simulink model "Protection"  (R2023b)
settings: Solver=FixedStepDiscrete  StartTime=0.0  StopTime=10.0  FixedStep=1e-4  RelTol=1e-3
undefined symbols (not defined in the file): PROTECTION_STATUS
libraries: simulink x5
settings Model: DataDictionary=Protection.sldd  Creator=84339  LastModifiedBy=84339
settings OptimizationCC: DefaultParameterBehavior=Inlined  EnhancedBackFolding=on  PassReuseOutputArgsAs=Individual arguments  ZeroExternalMemoryAtStartup=off  ZeroInternalMemoryAtStartup=off  OptimizeBlockOrder=speed  DifferentSizesBufferReuse=on  OptimizationCustomize=off  EfficientTunableParamExpr=on
settings DebuggingCC: ParameterTunabilityLossMsg=error
settings SFSimCC: MATLABDynamicMemAlloc=off
settings RTWCC: Description=Embedded Coder  SystemTargetFile=ert.tlc  EmbeddedCoderDictionary=Arch.sldd  GenCodeOnly=on  TemplateMakefile=ert_default_tmf
settings CodeAppCC: ForceParamTrailComments=on  IgnoreCustomStorageClasses=off  OperatorAnnotations=on  SimulinkDataObjDesc=on  SFDataObjDesc=on  InsertBlockDesc=on
settings ERTTargetCC: TargetLangStandard=C99 (ISO)  GenerateSampleERTMain=on  InlinedParameterPlacement=NonHierarchical  ERTCustomFileTemplate=example_file_process.tlc

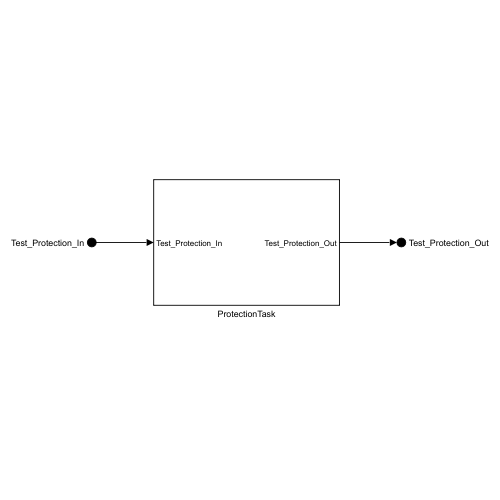
[thumbnail: Simulink's stored preview of the top-level diagram]
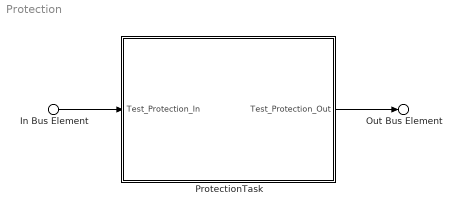
== system Protection ==
  In Bus Element : Inport  PortName=Test_Protection_In
  ProtectionTask : Subsystem
  Out Bus Element : Outport  PortName=Test_Protection_Out
  wires:
  In Bus Element/1 -> ProtectionTask/1(Test_Protection_In)
  ProtectionTask/1(Test_Protection_Out) -> Out Bus Element/1

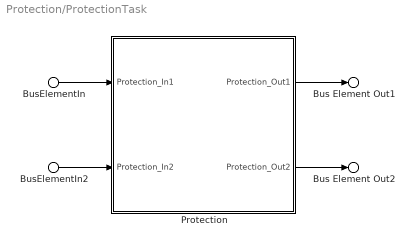
== system Protection/ProtectionTask ==
  BusElementIn : Inport  PortName=Test_Protection_In  Element=Protection_In1
  BusElementIn2 : Inport  PortName=Test_Protection_In  Element=Protection_In2
  Protection : Subsystem
  Bus Element Out1 : Outport  PortName=Test_Protection_Out  Element=Protection_Out1
  Bus Element Out2 : Outport  PortName=Test_Protection_Out  Element=Protection_Out2
  wires:
  BusElementIn/1 -> Protection/1(Protection_In1)
  Protection/1(Protection_Out1) -> Bus Element Out1/1
  BusElementIn2/1 -> Protection/2(Protection_In2)
  Protection/2(Protection_Out2) -> Bus Element Out2/1

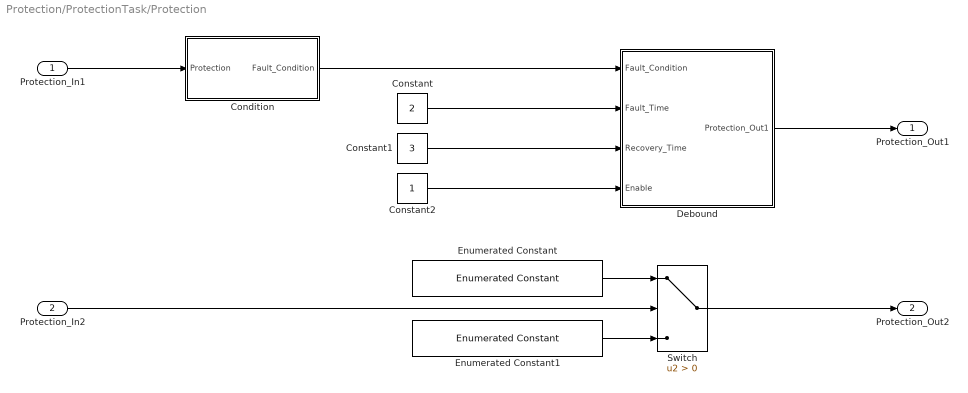
== system Protection/ProtectionTask/Protection ==
  Protection_In1 : Inport
  Protection_In2 : Inport  Port=2
  Condition : Subsystem
  Constant : Constant  Value=2  OutDataTypeStr=single
  Constant1 : Constant  Value=3  OutDataTypeStr=single
  Constant2 : Constant  OutDataTypeStr=boolean
  Debound : Subsystem
  Enumerated Constant : simulink/Sources/Enumerated Constant  OutDataTypeStr=Enum: PROTECTION_STATUS  Value=PROTECTION_STATUS.NORMAL  SampleTime=-1
  Enumerated Constant1 : simulink/Sources/Enumerated Constant  OutDataTypeStr=Enum: PROTECTION_STATUS  Value=PROTECTION_STATUS.ERROR  SampleTime=-1
  Switch : Switch  Criteria=u2 > Threshold  SaturateOnIntegerOverflow=off  InputSameDT=off
  Protection_Out1 : Outport
  Protection_Out2 : Outport  Port=2
  wires:
  Constant/1 -> Debound/2(Fault_Time)
  Constant1/1 -> Debound/3(Recovery_Time)
  Constant2/1 -> Debound/4(Enable)
  Debound/1(Protection_Out1) -> Protection_Out1/1
  Protection_In1/1 -> Condition/1(Protection)
  Condition/1(Fault_Condition) -> Debound/1(Fault_Condition)
  Protection_In2/1 -> Switch/2
  Enumerated Constant/1 -> Switch/1
  Enumerated Constant1/1 -> Switch/3
  Switch/1 -> Protection_Out2/1

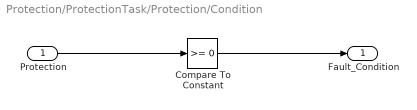
== system Protection/ProtectionTask/Protection/Condition ==
  Protection : Inport
  Compare To Constant : simulink/Logic and Bit Operations/Compare To Constant  relop=>=  const=0  OutDataTypeStr=boolean
  Fault_Condition : Outport
  wires:
  Compare To Constant/1 -> Fault_Condition/1
  Protection/1 -> Compare To Constant/1

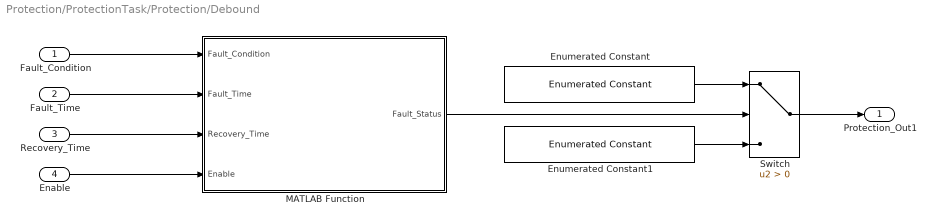
== system Protection/ProtectionTask/Protection/Debound ==
  Fault_Condition : Inport
  Fault_Time : Inport  Port=2
  Recovery_Time : Inport  Port=3
  Enable : Inport  Port=4
  Enumerated Constant : simulink/Sources/Enumerated Constant  OutDataTypeStr=Enum: PROTECTION_STATUS  Value=PROTECTION_STATUS.NORMAL  SampleTime=-1
  Enumerated Constant1 : simulink/Sources/Enumerated Constant  OutDataTypeStr=Enum: PROTECTION_STATUS  Value=PROTECTION_STATUS.ERROR  SampleTime=-1
  MATLAB Function : MATLAB Function  TreatAsAtomicUnit=on
  Switch : Switch  Criteria=u2 > Threshold  SaturateOnIntegerOverflow=off  InputSameDT=off
  Protection_Out1 : Outport
  wires:
  Enumerated Constant1/1 -> Switch/3
  MATLAB Function/1(Fault_Status) -> Switch/2
  Switch/1 -> Protection_Out1/1
  Enumerated Constant/1 -> Switch/1
  Fault_Condition/1 -> MATLAB Function/1(Fault_Condition)
  Fault_Time/1 -> MATLAB Function/2(Fault_Time)
  Recovery_Time/1 -> MATLAB Function/3(Recovery_Time)
  Enable/1 -> MATLAB Function/4(Enable)

== matlab function Protection/ProtectionTask/Protection/Debound/MATLAB Function ==
  data: Fault_Condition input; Fault_Status output; Fault_Time input; Recovery_Time input; Enable input
function Fault_Status = Debounce_Function(Fault_Condition, Fault_Time, Recovery_Time, Enable)
%#codegen

persistent Fault_Timer;
persistent Recovery_Timer;
persistent Fault_Active;

if isempty(Fault_Timer)
    Fault_Timer = single(0.0);
    Recovery_Timer = single(0.0);
    Fault_Active = false;
end

Ts = single(0.01);  % 10ms

if ~Enable
    Fault_Timer = single(0.0);
    Recovery_Timer = single(0.0);
    Fault_Active = false;

else
    if ~Fault_Active

        % Fault detection
        if Fault_Condition
            Fault_Timer = Fault_Timer + Ts;
        else
            Fault_Timer = single(0.0);
        end

        if Fault_Timer >= single(Fault_Time)
            Fault_Active = true;
            Recovery_Timer = single(0.0);
        end

    else

        % Fault recovery
        if ~Fault_Condition
            Recovery_Timer = Recovery_Timer + Ts;
        else
            Recovery_Timer = single(0.0);
        end

        if Recovery_Timer >= single(Recovery_Time)
            Fault_Active = false;
            Fault_Timer = single(0.0);
        end

    end
end

Fault_Status = Fault_Active;

end
